simulink model "ps5_openloop_identification_2ms_UPDATED"  (R2024a)
settings: Solver=FixedStepDiscrete  StartTime=0.0  StopTime=10  FixedStep=0.002  RelTol=1e-3
model workspace (MAT data in the model file):
  staircase_data = [0 0.002 0.004 0.006 0.008 0.01 0.012 0.014 0.016 0.018 0.02 0.022 ... (10002 elements, 5001x2)]
settings Model: Creator=tanuj  LastModifiedBy=tanuj
settings DataIOCC: SaveFormat=Array  TimeSaveName=t

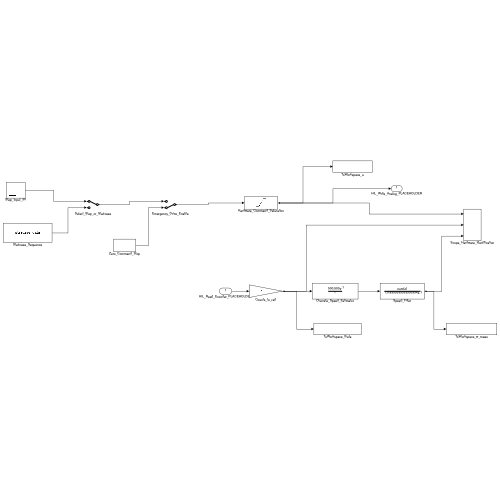
[thumbnail: Simulink's stored preview of the top-level diagram]
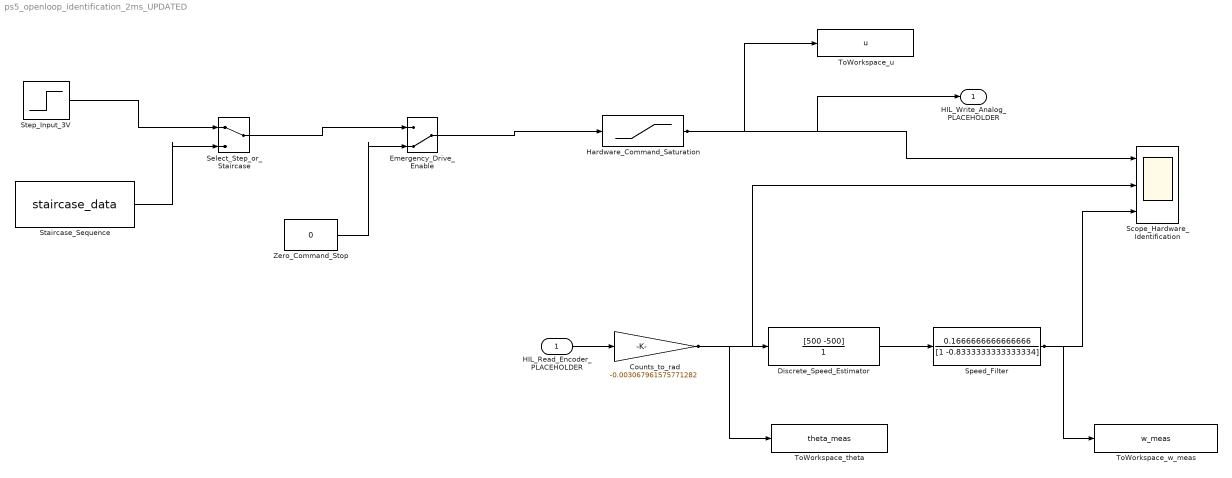
== system ps5_openloop_identification_2ms_UPDATED ==
  HIL_Read_Encoder_PLACEHOLDER : Inport
  Counts_to_rad : Gain  Gain=-0.003067961575771282
  Discrete_Speed_Estimator : DiscreteFilter  Numerator=[500 -500]  Denominator=1  SampleTime=0.002
  Emergency_Drive_Enable : ManualSwitch  CurrentSetting=0
  Hardware_Command_Saturation : Saturate  UpperLimit=10  LowerLimit=-10
  Scope_Hardware_Identification : Scope  NumInputPorts=3
  Select_Step_or_Staircase : ManualSwitch
  Speed_Filter : DiscreteFilter  Numerator=0.1666666666666666  Denominator=[1 -0.8333333333333334]  SampleTime=0.002
  Staircase_Sequence : FromWorkspace  VariableName=staircase_data  Interpolate=off
  Step_Input_3V : Step  Time=0.5  After=3  SampleTime=0.002
  ToWorkspace_theta : ToWorkspace  VariableName=theta_meas  SampleTime=-1
  ToWorkspace_u : ToWorkspace  VariableName=u  SampleTime=-1
  ToWorkspace_w_meas : ToWorkspace  VariableName=w_meas  SampleTime=-1
  Zero_Command_Stop : Constant  Value=0  SampleTime=0.002
  HIL_Write_Analog_PLACEHOLDER : Outport
  wires:
  Step_Input_3V/1 -> Select_Step_or_Staircase/1
  Staircase_Sequence/1 -> Select_Step_or_Staircase/2
  Select_Step_or_Staircase/1 -> Emergency_Drive_Enable/1
  Zero_Command_Stop/1 -> Emergency_Drive_Enable/2
  Emergency_Drive_Enable/1 -> Hardware_Command_Saturation/1
  Hardware_Command_Saturation/1 -> HIL_Write_Analog_PLACEHOLDER/1, ToWorkspace_u/1, Scope_Hardware_Identification/1
  HIL_Read_Encoder_PLACEHOLDER/1 -> Counts_to_rad/1
  Counts_to_rad/1 -> Discrete_Speed_Estimator/1, ToWorkspace_theta/1, Scope_Hardware_Identification/2
  Discrete_Speed_Estimator/1 -> Speed_Filter/1
  Speed_Filter/1 -> ToWorkspace_w_meas/1, Scope_Hardware_Identification/3
